simulink model "test_on_proxy"  (R2025b)
settings: Solver=FixedStepAuto  StartTime=0.0  StopTime=91  FixedStep=0.001  RelTol=1e-3
undefined symbols (not defined in the file): DiscIntNeverNeededParam, Ts, x0_eq
libraries: eeGeneralControl x1
(part 1 of 2)
settings Model: Creator=Juuzo  LastModifiedBy=Juuzo
settings SolverCC: AlgebraicLoopSolver=TrustRegion
settings SFSimCC: CustomCodeUndefinedFunction=UseInterfaceOnly
settings RTWCC: GPUComputeCapability=3.5

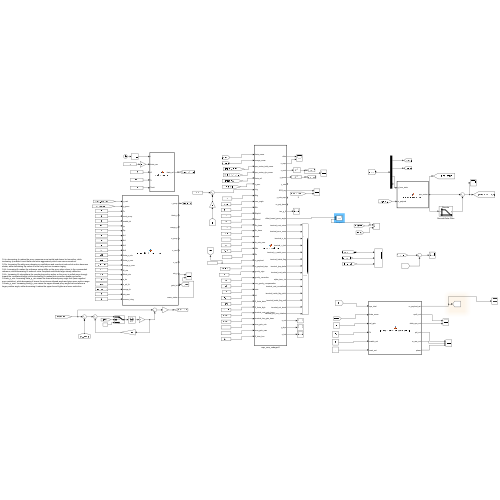
[thumbnail: Simulink's stored preview of the top-level diagram]
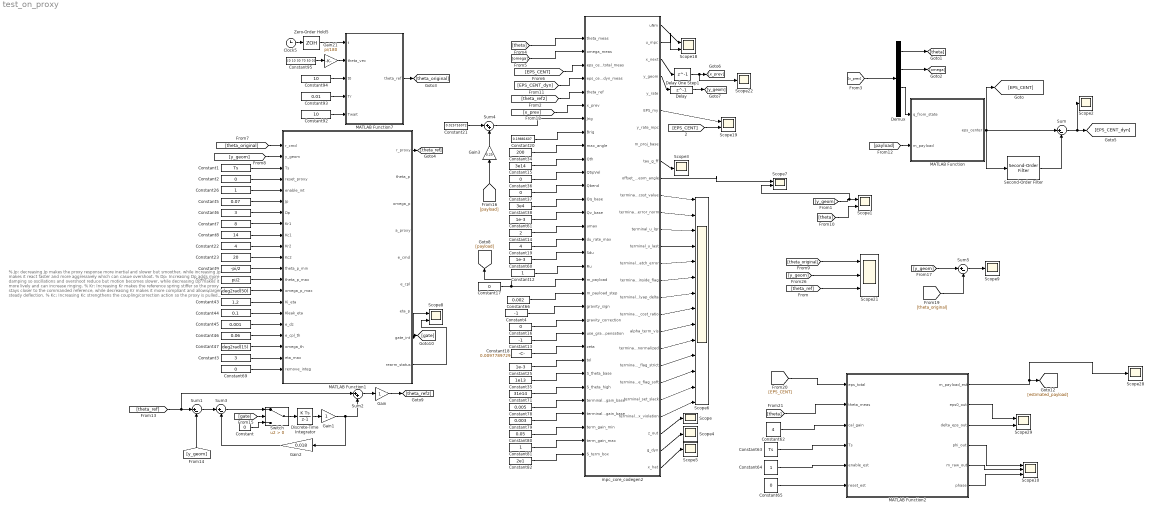
== system test_on_proxy ==
  note: % Jp: decreasing Jp makes the proxy response more inertial and slower but smoother, while increasing Jp makes it react faster and more aggressively which can casue overshoot.
      | % Dp: Increasing Dp adds more damping so oscillations and overshoot reduce but motion becomes slower, while decreasing Dp makes it more lively and can increase ringing.
      | % Kr: Increasing Kr makes the reference spring stiffer so the proxy stays closer to the commanded reference, while decreasing Kr makes it more compliant and allows larger steady deflection.
      | % Kc: Increasing Kc strengthens the coupling/correction action so the proxy is pulled more strongly toward the constrained target, while decreasing Kc makes that correction weaker and softer.
      | % theta_p_min: Increasing theta_p_min raises the lower allowed proxy angle limit (less negative / more restrictive), while decreasing it lowers the minimum allowed angle and gives more motion range.
      | % theta_p_max: Increasing theta_p_max raises the upper allowed proxy angle limit and allows a larger positive angle, while decreasing it makes the upper bound tighter and more restrictive.
  Clock5 : Clock
  Constant{,2,16..17,37,65,69} (7 alike) : Constant  Value=0
  Constant1 : Constant  Value=Ts
  Constant10 : Constant  Value=deg2rad(50)
  Constant11 : Constant  Value=pi/2
  Constant12 : Constant
  Constant13 : Constant  Value=-1
  Constant14 : Constant  Value=2
  Constant15 : Constant  Value=3e14  VectorParams1D=off
  Constant18 : Constant  Value=0.0097789729
  Constant19 : Constant  Value=4
  Constant20 : Constant  Value=0.19881607
  Constant21 : Constant  Value=0.025755072
  Constant22 : Constant  Value=4
  Constant23 : Constant  Value=20
  Constant25 : Constant  Value=1e-3
  Constant26 : Constant  VectorParams1D=off
  Constant3 : Constant  Value=3
  Constant34 : Constant  Value=200
  Constant35 : Constant  Value=1e13
  Constant36 : Constant  Value=0  VectorParams1D=off
  Constant38 : Constant  Value=3e4  VectorParams1D=off
  Constant4 : Constant  Value=-1
  Constant43 : Constant  Value=1.2
  Constant44 : Constant  Value=0.1
  Constant45 : Constant  Value=0.001
  Constant46 : Constant  Value=0.06
  Constant47 : Constant  Value=deg2rad(15)
  Constant5 : Constant  Value=0.07
  Constant6 : Constant  Value=3
  Constant60 : Constant  Value=1e-3
  Constant61 : Constant  Value=1e-3
  Constant62 : Constant  Value=4
  Constant63 : Constant  Value=Ts
  Constant64 : Constant
  Constant66 : Constant  Value=0.002
  Constant7 : Constant  Value=8
  Constant71 : Constant  Value=31e14
  Constant78 : Constant  Value=0.005
  Constant79 : Constant  Value=0.003
  Constant8 : Constant  Value=14
  Constant80 : Constant  Value=0.05
  Constant81 : Constant
  Constant82 : Constant  Value=2e1
  Constant9 : Constant  Value=-pi/2
  Constant92 : Constant  Value=10
  Constant93 : Constant  Value=0.01
  Constant94 : Constant  Value=10
  Constant95 : Constant  Value=[0 10 30 70 50 0]  VectorParams1D=off
  Delay : Delay  DelayLength=1
  Delay One Step1 : Delay  DelayLength=1  InitialCondition=[-0.4 0 0 0]  SampleTime=Ts
  Demux : Demux  Outputs=size(x0_eq,1)
  Discrete-Time Integrator : DiscreteIntegrator  SampleTime=-1  ICPrevOutput=DiscIntNeverNeededParam  ICPrevScaledInput=DiscIntNeverNeededParam
  Gain : Gain
  Gain1 : Gain
  Gain2 : Gain  Gain=0.018
  Gain21 : Gain  Gain=pi/180
  Gain3 : Gain  Gain=0.25
  MATLAB Function : MATLAB Function  TreatAsAtomicUnit=on
  MATLAB Function1 : MATLAB Function  TreatAsAtomicUnit=on
  MATLAB Function2 : MATLAB Function  TreatAsAtomicUnit=on  SystemSampleTime=0.001
  MATLAB Function7 : MATLAB Function  TreatAsAtomicUnit=on
  Scope{,2..5,9,22,28} (8 alike) : Scope
      Scope settings: ActiveDisplayYMinimum=0.03462626429758181  ActiveDisplayYMaximum=0.14630000608700439
      Scope2 settings: ActiveDisplayYMinimum=-2.6432719878301515E-6  ActiveDisplayYMaximum=1.0572577019271434E-6  DataLoggingVariableName=ScopeData2
      Scope22 settings: ActiveDisplayYMinimum=-0.0014754347139640661  ActiveDisplayYMaximum=0.0005793847718010294  DataLoggingVariableName=ScopeData7
      Scope28 settings: ActiveDisplayYMinimum=-0.00425  ActiveDisplayYMaximum=0.03825  DataLoggingVariableName=ScopeData15
      Scope3 settings: ActiveDisplayYMinimum=-1  ActiveDisplayYMaximum=1  DataLoggingVariableName=ScopeData5
      Scope4 settings: ActiveDisplayYMinimum=0.03462626429758181  ActiveDisplayYMaximum=0.14630000608700439  DataLoggingVariableName=ScopeData8
      Scope5 settings: ActiveDisplayYMinimum=0.03462626429758181  ActiveDisplayYMaximum=0.14630000608700439  DataLoggingVariableName=ScopeData9
      Scope9 settings: ActiveDisplayYMinimum=-0.00729154121661256  ActiveDisplayYMaximum=0.005693566274452444  DataLoggingVariableName=ScopeData13
  Scope{1,7..8,18..19,29} (6 alike) : Scope  NumInputPorts=2
      Scope1 settings: ActiveDisplayYMinimum=-1  ActiveDisplayYMaximum=1
      Scope18 settings: ActiveDisplayYMinimum=-2.5  ActiveDisplayYMaximum=2.5  DataLoggingVariableName=ScopeData3
      Scope19 settings: ActiveDisplayYMinimum=-4.4042134344337806E+284  ActiveDisplayYMaximum=1.9921108400400171E+284  DataLoggingVariableName=ScopeData4
      Scope29 settings: ActiveDisplayYMinimum=6.3875  ActiveDisplayYMaximum=6.5125  DataLoggingVariableName=ScopeData16
      Scope7 settings: ActiveDisplayYMinimum=-0.00025935118136851537  ActiveDisplayYMaximum=0.007136419000205705  DataLoggingVariableName=ScopeData11
      Scope8 settings: ActiveDisplayYMinimum=-0.12499999999999997  ActiveDisplayYMaximum=1.125  DataLoggingVariableName=ScopeData12
  Scope10 : Scope  NumInputPorts=3
      settings: ActiveDisplayYMinimum=-0.06335  ActiveDisplayYMaximum=0.08278  DataLoggingVariableName=ScopeData14
  Scope21 : Scope  NumInputPorts=3
      settings: ActiveDisplayYMinimum=-0.60273685089963092  ActiveDisplayYMaximum=1.4244490683177709  DataLoggingVariableName=ScopeData6
  Scope6 : Scope  NumInputPorts=14
      settings: ActiveDisplayYMinimum=-1  ActiveDisplayYMaximum=1  DataLoggingVariableName=ScopeData10
  Second-Order Filter : eeGeneralControl/Second-Order Filter  FilterType=Low-pass  fn=25  Zeta=0.707  Ts=-1  A0=0  Ph0=0  f0=0  b0=0
      settings: LibrarySourceBlock=ee_sl_lib/General Control/Second-Order Filter
  Sum{,1,3,5} (4 alike) : Sum  Inputs=|+-
  Sum2 : Sum  Inputs=|++
  Sum4 : Sum  Inputs=|++
  Switch : Switch  Criteria=u2 > Threshold  SaturateOnIntegerOverflow=off  InputSameDT=off
  Zero-Order Hold5 : ZeroOrderHold  SampleTime=Ts
  mpc_core_codegen2 : MATLAB Function  TreatAsAtomicUnit=on  SystemSampleTime=Ts
  wires:
  [x_prev] -> Demux/1
  Constant93/1 -> MATLAB Function7/4(Tr)
  Gain21/1 -> MATLAB Function7/2(theta_vec)
  Zero-Order Hold5/1 -> MATLAB Function7/1(t)
  Clock5/1 -> Zero-Order Hold5/1
  Constant94/1 -> MATLAB Function7/3(t0)
  Constant92/1 -> MATLAB Function7/5(Twait)
  [EPS_CENT] -> Scope19/2
  Constant95/1 -> Gain21/1
  [theta_original] -> MATLAB Function1/1(r_cmd)
  [y_geom] -> MATLAB Function1/2(y_geom)
  MATLAB Function7/1(theta_ref) -> [theta_original]
  MATLAB Function1/1(r_proxy) -> [theta_ref]
  Demux/3 -> MATLAB Function/1(q_from_state)
  Demux/1 -> [theta]
  Demux/2 -> [omega]
  MATLAB Function/1(eps_center) -> Second-Order Filter/1, Sum/1, [EPS_CENT]
  Delay/1 -> [y_geom]
  [theta_original] -> Scope21/1
  [theta_ref] -> Scope21/3
  Delay One Step1/1 -> Scope22/1, [x_prev]
  [y_geom] -> Scope21/2
  [y_geom] -> Scope7/2, Scope1/1
  [theta] -> Scope1/2
  [theta] -> mpc_core_codegen2/1(theta_meas)
  [omega] -> mpc_core_codegen2/2(omega_meas)
  [EPS_CENT] -> mpc_core_codegen2/3(eps_center_total_meas)
  Constant20/1 -> mpc_core_codegen2/8(Brig)
  [x_prev] -> mpc_core_codegen2/6(x_prev)
  [theta_ref2] -> mpc_core_codegen2/5(theta_ref)
  Second-Order Filter/1 -> Sum/2
  Sum/1 -> Scope2/1, [EPS_CENT_dyn]
  mpc_core_codegen2/1(uNm) -> Scope18/1
  mpc_core_codegen2/2(u_mpc) -> Scope18/2
  mpc_core_codegen2/3(x_next) -> Delay One Step1/1
  mpc_core_codegen2/4(y_geom) -> Delay/1
  [payload] -> MATLAB Function/2(m_payload)
  mpc_core_codegen2/6(EPS_my) -> Scope19/1
  mpc_core_codegen2/9(tau_g_ff) -> Scope3/1
  mpc_core_codegen2/25(z_out) -> Scope/1
  mpc_core_codegen2/26(g_dyn) -> Scope4/1
  mpc_core_codegen2/27(x_hat) -> Scope5/1
  mpc_core_codegen2/10(offset_based_geom_angle) -> Scope7/1
  mpc_core_codegen2/11(terminal_cost_value) -> Scope6/1
  mpc_core_codegen2/12(terminal_error_norm) -> Scope6/2
  mpc_core_codegen2/13(terminal_u_lqr) -> Scope6/3
  mpc_core_codegen2/14(terminal_u_last) -> Scope6/4
  mpc_core_codegen2/15(terminal_u_match_error) -> Scope6/5
  mpc_core_codegen2/16(terminal_inside_flag) -> Scope6/6
  mpc_core_codegen2/17(terminal_lyap_delta) -> Scope6/7
  mpc_core_codegen2/18(terminal_cost_ratio) -> Scope6/8
  mpc_core_codegen2/19(alpha_term_vis) -> Scope6/9
  mpc_core_codegen2/20(terminal_cost_normalized) -> Scope6/10
  mpc_core_codegen2/21(terminal_inside_flag_strict) -> Scope6/11
  mpc_core_codegen2/22(terminal_inside_flag_soft) -> Scope6/12
  mpc_core_codegen2/23(terminal_set_slack) -> Scope6/13
  mpc_core_codegen2/24(terminal_set_box_violation) -> Scope6/14
  [theta_ref] -> Sum2/1, Sum1/1
  [y_geom] -> Sum1/2
  Sum2/1 -> Gain/1
  Gain/1 -> [theta_ref2]
  [gate] -> Switch/2
  MATLAB Function1/8(gate_int) -> [gate], Scope8/1
  Constant/1 -> Switch/3
  Sum1/1 -> Sum3/1
  Sum3/1 -> Switch/1
  Switch/1 -> Discrete-Time Integrator/1
  Discrete-Time Integrator/1 -> Gain1/1
  Gain1/1 -> Sum2/2, Gain2/1
  Gain2/1 -> Sum3/2
  Constant21/1 -> Sum4/1
  [payload] -> Gain3/1
  Sum4/1 -> mpc_core_codegen2/7(Jrig)
  Gain3/1 -> Sum4/2
  MATLAB Function1/9(rearm_status) -> Scope8/2
  [y_geom] -> Sum5/1
  [theta_original] -> Sum5/2
  Sum5/1 -> Scope9/1
  [EPS_CENT_dyn] -> mpc_core_codegen2/4(eps_center_dyn_meas)
  Constant63/1 -> MATLAB Function2/4(Ts)
  MATLAB Function2/6(phase) -> Scope10/3
  [theta] -> MATLAB Function2/2(theta_meas)
  MATLAB Function2/4(phi_out) -> Scope10/1
  [EPS_CENT] -> MATLAB Function2/1(eps_total)
  Constant65/1 -> MATLAB Function2/6(reset_est)
  MATLAB Function2/5(m_raw_out) -> Scope10/2
  MATLAB Function2/3(delta_eps_out) -> Scope29/2
  MATLAB Function2/2(eps0_out) -> Scope29/1
  MATLAB Function2/1(m_payload_est) -> Scope28/1, [estimated_payload]
  Constant64/1 -> MATLAB Function2/5(enable_est)
  Constant62/1 -> MATLAB Function2/3(cal_gain)
  Constant12/1 -> mpc_core_codegen2/18(Ru)
  Constant36/1 -> mpc_core_codegen2/11(QtipVel)
  Constant13/1 -> mpc_core_codegen2/23(use_gravity_compensation)
  Constant71/1 -> mpc_core_codegen2/27(S_theta_high)
  Constant25/1 -> mpc_core_codegen2/25(tol)
  Constant79/1 -> mpc_core_codegen2/29(terminal_law_gain_base)
  Constant15/1 -> mpc_core_codegen2/10(Qth)
  Constant60/1 -> mpc_core_codegen2/17(Sdu)
  Constant66/1 -> mpc_core_codegen2/20(m_payload_step)
  Constant78/1 -> mpc_core_codegen2/28(terminal_cost_gain_base)
  Constant38/1 -> mpc_core_codegen2/13(Qq_base)
  Constant4/1 -> mpc_core_codegen2/21(gravity_sign)
  Constant16/1 -> mpc_core_codegen2/22(gravity_correction)
  Constant18/1 -> mpc_core_codegen2/24(zeta)
  Constant80/1 -> mpc_core_codegen2/30(term_gain_min)
  Constant35/1 -> mpc_core_codegen2/26(S_theta_base)
  Constant19/1 -> mpc_core_codegen2/16(du_rate_max)
  Constant14/1 -> mpc_core_codegen2/15(umax)
  Constant61/1 -> mpc_core_codegen2/14(Qv_base)
  Constant34/1 -> mpc_core_codegen2/9(max_angle)
  Constant37/1 -> mpc_core_codegen2/12(Qbend)
  Constant82/1 -> mpc_core_codegen2/32(S_term_box)
  Constant81/1 -> mpc_core_codegen2/31(term_gain_max)
  Constant17/1 -> mpc_core_codegen2/19(m_payload), [payload]
  Constant7/1 -> MATLAB Function1/8(Kr1)
  Constant46/1 -> MATLAB Function1/18(e_cpl_th)
  Constant8/1 -> MATLAB Function1/9(Kc1)
  Constant10/1 -> MATLAB Function1/14(omega_p_max)
  Constant9/1 -> MATLAB Function1/12(theta_p_min)
  Constant23/1 -> MATLAB Function1/11(Kc2)
  Constant11/1 -> MATLAB Function1/13(theta_p_max)
  Constant47/1 -> MATLAB Function1/19(omega_th)
  Constant26/1 -> MATLAB Function1/5(enable_int)
  Constant44/1 -> MATLAB Function1/16(Kleak_eta)
  Constant2/1 -> MATLAB Function1/4(reset_proxy)
  Constant22/1 -> MATLAB Function1/10(Kr2)
  Constant1/1 -> MATLAB Function1/3(Ts)
  Constant5/1 -> MATLAB Function1/6(Jp)
  Constant43/1 -> MATLAB Function1/15(Ki_eta)
  Constant3/1 -> MATLAB Function1/20(eta_max)
  Constant69/1 -> MATLAB Function1/21(remove_integ)
  Constant45/1 -> MATLAB Function1/17(e_dz)
  Constant6/1 -> MATLAB Function1/7(Dp)

== matlab function test_on_proxy/MATLAB Function1 ==
  data: r_cmd input; r_proxy output; y_geom input; Ts input; reset_proxy input; enable_int input; Jp input; Dp input; Kr1 input; Kc1 input; Kr2 input; Kc2 input; theta_p_min input; theta_p_max input; omega_p_max input; theta_p output; omega_p output; a_proxy output; e_cmd output; e_cpl output; Ki_eta input; Kleak_eta input; e_dz input; e_cpl_th input; omega_th input; eta_max input; eta_p output; gate_int output; remove_integ input; rearm_status output
function [r_proxy, theta_p, omega_p, a_proxy, e_cmd, e_cpl, eta_p, gate_int,rearm_status] = proxy_virtual_beam_int_strict( ...
    r_cmd, y_geom, Ts, reset_proxy, enable_int, ...
    Jp, Dp, Kr1, Kc1, Kr2, Kc2, ...
    theta_p_min, theta_p_max, omega_p_max, ...
    Ki_eta, Kleak_eta, e_dz, e_cpl_th, omega_th, eta_max,remove_integ) %#codegen

persistent thp wpp etap init_done
persistent int_armed
persistent r_cmd_prev
persistent soft_mode
persistent abs_e_prev err_dec_count
persistent e_bias_prev

if isempty(init_done)
    thp = 0.0;
    wpp = 0.0;
    etap = 0.0;
    int_armed = 1.0;
    r_cmd_prev = r_cmd;
    soft_mode = 0.0;
    abs_e_prev = 0.0;
    err_dec_count = 0.0;
    e_bias_prev = 0.0;
    init_done = true;
end

if reset_proxy ~= 0
    thp  = 0.0;
    wpp  = 0.0;
    etap = 0.0;
    int_armed = 1.0;
    r_cmd_prev = r_cmd;
    soft_mode = 0.0;
    abs_e_prev = 0.0;
    err_dec_count = 0.0;
    e_bias_prev = 0.0;
end

Ts_eff      = max(Ts, 1e-9);
Jp_eff      = max(Jp, 1e-9);
wmax        = max(omega_p_max, 1e-9);
eta_lim     = max(abs(eta_max), 1e-9);

e_dead      = max(abs(e_dz), 0.0);
e_act       = max(abs(e_cpl_th), e_dead + 1e-9);

% smarter / earlier rearm than previous 2.0*e_act
e_rearm     = 1.2 * e_act;

omega_lim   = max(abs(omega_th), 0.0);

% -------------------------------------------------------------------------
% command-change detection
% if original reference changes, leave soft mode immediately
% -------------------------------------------------------------------------
r_move_th = 0.1*pi/180.0;
r_changed = abs(r_cmd - r_cmd_prev) >= r_move_th;
r_is_static = ~r_changed;

if r_changed
    soft_mode = 0.0;
    int_armed = 1.0;
    err_dec_count = 0.0;
    e_bias_prev = 0.0;
end

% -------------------------------------------------------------------------
% current coupling error between proxy and real beam
% positive if proxy is ahead of the real beam
% -------------------------------------------------------------------------
e_cpl_k = thp - y_geom;

% -------------------------------------------------------------------------
% bias error for integral action
% -------------------------------------------------------------------------
e_bias = r_cmd - y_geom;
abs_e_bias = abs(e_bias);

% -------------------------------------------------------------------------
% release detection while in soft mode
% if error is decreasing for several samples, assume beam was released
% and return to normal stiffness so it comes back faster
% -------------------------------------------------------------------------
N_dec_required = 10.0;
e_dec_tol = 0.02*pi/180.0;

if soft_mode ~= 0.0
    if abs_e_bias < (abs_e_prev - e_dec_tol)
        err_dec_count = err_dec_count + 1.0;
    else
        err_dec_count = 0.0;
    end

    if err_dec_count >= N_dec_required
        soft_mode = 0.0;
        err_dec_count = 0.0;
    end
else
    err_dec_count = 0.0;
end

abs_e_prev = abs_e_bias;

% -------------------------------------------------------------------------
% smarter integral arming logic
%
% old problem:
%   if error entered deadzone during overshoot, integral was disarmed
%   and stayed off until abs(error) reached a large rearm threshold.
%
% new idea:
%   disarm only if close to reference AND not moving away.
%   if error crossed sign or starts growing again, keep/rearm integral.
% -------------------------------------------------------------------------
e_dot_est = (e_bias - e_bias_prev) / Ts_eff;

% true if error magnitude is increasing
moving_away = (e_bias * e_dot_est) > 0.0;

% true if beam crossed the reference
sign_crossed = (e_bias * e_bias_prev) < 0.0;

if abs_e_bias <= e_dead
    if moving_away || sign_crossed
        int_armed = 1.0;
    else
        int_armed = 0.0;
    end
elseif abs_e_bias >= e_act
    int_armed = 1.0;
end
rearm_status = int_armed;
% -------------------------------------------------------------------------
% final strict integral gate
% allow integral action up to e_rearm for overshoot recovery
% -------------------------------------------------------------------------
if (enable_int ~= 0) && ...
   (int_armed ~= 0) && ...
   (abs_e_bias > e_dead) && ...
   (abs_e_bias <= e_rearm) && ...
   (abs(wpp) <= omega_lim)
    gate = 1.0;
else
    gate = 0.0;
end

% -------------------------------------------------------------------------
% latch soft/compliant mode
%
% enter soft mode only when:
%   1) command is constant
%   2) beam is fully close to reference, inside deadband
%   3) proxy is moving slowly
%   4) integral gate is already off
%
% once soft_mode = 1, keep it no matter gate changes,
% until r_cmd changes or release detection switches it back.
% -------------------------------------------------------------------------
near_dead  = abs_e_bias <= e_dead;
proxy_slow = abs(wpp) <= omega_lim;

if (soft_mode == 0.0) && r_is_static && near_dead && proxy_slow && (gate == 0.0)
    soft_mode = 1.0;
end

if soft_mode ~= 0.0
    Kr_eff = Kr2;
    Kc_eff = Kc2;
else
    Kr_eff = Kr1;
    Kc_eff = Kc1;
end

e_bias_dz = deadzone_scalar(e_bias, e_dead);

% -------------------------------------------------------------------------
% internal integral bias state
% if gate = 0, eta is frozen
% -------------------------------------------------------------------------
if gate ~= 0
    eta_dot = Ki_eta * e_bias_dz - Kleak_eta * etap;
else
    eta_dot = 0.0;
end

etap = etap + Ts_eff * eta_dot;
etap = clamp_scalar(etap, -eta_lim, eta_lim);

% -------------------------------------------------------------------------
% command-side spring error
% -------------------------------------------------------------------------
e_cmd_k = (r_cmd + remove_integ*etap) - thp;

% -------------------------------------------------------------------------
% proxy rigid-body dynamics
% -------------------------------------------------------------------------
w_dot = (-Dp*wpp + Kr_eff*e_cmd_k - Kc_eff*e_cpl_k) / Jp_eff;

wpp = wpp + Ts_eff * w_dot;
wpp = clamp_scalar(wpp, -wmax, wmax);

thp = thp + Ts_eff * wpp;
thp = clamp_scalar(thp, theta_p_min, theta_p_max);

if (thp <= theta_p_min) && (wpp < 0.0)
    wpp = 0.0;
elseif (thp >= theta_p_max) && (wpp > 0.0)
    wpp = 0.0;
end

% update memories
r_cmd_prev = r_cmd;
e_bias_prev = e_bias;

r_proxy  = thp;
theta_p  = thp;
omega_p  = wpp;
a_proxy  = w_dot;
e_cmd    = e_cmd_k;
e_cpl    = e_cpl_k;
eta_p    = etap;
gate_int = gate;

end

function y = clamp_scalar(x, xmin, xmax)
y = min(max(x, xmin), xmax);
end

function y = deadzone_scalar(x, dz)
if abs(x) <= dz
    y = 0.0;
elseif x > dz
    y = x - dz;
else
    y = x + dz;
end
end

== matlab function test_on_proxy/MATLAB Function ==
  data: q_from_state input; eps_center output; m_payload input
function eps_center = eps_from_state_block(q_from_state, m_payload)
%#codegen
% Standalone strain generator from modal state q1
%
% Input:
%   q_from_state : modal coordinate q1
%   m_payload    : payload mass at beam tip [kg]
%
% Output:
%   eps_center   : strain at sensor location
%
% Assumption:
%   payload rotational inertia J_tip = 0

persistent init_done last_m_payload k_strain

% --- required explicit initialization for MATLAB Function/codegen ---
if isempty(init_done)
    init_done = false;
    last_m_payload = 0.0;
    k_strain = 0.0;
end

need_rebuild = false;
if ~init_done
    need_rebuild = true;
elseif abs(last_m_payload - m_payload) > 1e-12
    need_rebuild = true;
end

if need_rebuild

    % ===== geometry & material =====
    L   = 0.5;
    b   = 0.02;
    h   = 0.002;
    E   = 70e9;
    rho = 2755;

    Acs  = b*h;
    Izz  = b*h^3/12;
    rhoA = rho*Acs;
    yb   = 0.5*h;

    % ===== payload =====
    M_tip = m_payload;
    J_tip = 0.0;

    % ===== spatial grid for normalization =====
    Ns = 100;
    s  = linspace(0, L, Ns).';

    w_trap = zeros(Ns,1);
    for i = 2:Ns
        hseg = s(i) - s(i-1);
        w_trap(i-1) = w_trap(i-1) + 0.5*hseg;
        w_trap(i)   = w_trap(i)   + 0.5*hseg;
    end

    % ===== first payload-aware root lambda = betaL =====
    betaL = compute_first_payload_root(rhoA, L, M_tip, J_tip);

    % ===== payload-aware shape =====
    phi_raw_tip = payload_shape_local(betaL, L, L, rhoA, M_tip);
    sc = 1 / max(abs(phi_raw_tip), 1e-12);

    phi_raw  = payload_shape_local(betaL, L, s, rhoA, M_tip) * sc;
    dphi_raw = payload_shape_d_local(betaL, L, s, rhoA, M_tip) * sc;

    % ===== payload-aware modal mass normalization =====
    mi = dot(w_trap, rhoA * (phi_raw.^2)) ...
       + M_tip * (phi_raw(end)^2) ...
       + J_tip * (dphi_raw(end)^2);

    cn = 1 / sqrt(max(mi, 1e-12));

    % ===== strain coefficient at sensor =====
    sensor_s = 0.05;

    phi_dd_i = payload_shape_dd_local(betaL, L, sensor_s, rhoA, M_tip);
    phi_dd_i = phi_dd_i * sc;

    psi_dd_i = cn * phi_dd_i;

    % epsilon = yb * psi_dd * q
    k_strain = yb * psi_dd_i;

    last_m_payload = m_payload;
    init_done = true;
end

eps_center = k_strain * q_from_state;

end

% ============================================================
% Helpers
% ============================================================

function betaL = compute_first_payload_root(rhoA, L, M_tip, J_tip)
% Finds first positive root of the payload-aware frequency equation
% in dimensionless variable lambda = beta * L

x_prev = 0.20;
f_prev = freq_eq_payload_lambda_local(x_prev, rhoA, L, M_tip, J_tip);

step = 0.02;
betaL = 1.875104068711961; % safe fallback

x = x_prev + step;
while x <= 10.0
    f_now = freq_eq_payload_lambda_local(x, rhoA, L, M_tip, J_tip);

    if isfinite(f_prev) && isfinite(f_now)
        if (f_prev * f_now) < 0
            betaL = bisect_payload_root_local(x_prev, x, rhoA, L, M_tip, J_tip);
            return;
        end
    end

    x_prev = x;
    f_prev = f_now;
    x = x + step;
end
end

function root = bisect_payload_root_local(a, b, rhoA, L, M_tip, J_tip)
fa = freq_eq_payload_lambda_local(a, rhoA, L, M_tip, J_tip);
fb = freq_eq_payload_lambda_local(b, rhoA, L, M_tip, J_tip);

if abs(fa) < 1e-12
    root = a;
    return;
end
if abs(fb) < 1e-12
    root = b;
    return;
end

for it = 1:80
    c = 0.5 * (a + b);
    fc = freq_eq_payload_lambda_local(c, rhoA, L, M_tip, J_tip);

    if abs(fc) < 1e-12 || abs(b - a) < 1e-10
        root = c;
        return;
    end

    if (fa * fc) < 0
        b = c;
        fb = fc;
    else
        a = c;
        fa = fc;
    end
end

root = 0.5 * (a + b);
end

function val = freq_eq_payload_lambda_local(lam, rhoA, L, M_tip, J_tip)
% Payload-aware frequency equation in dimensionless form:
%
% 1 + cos(lam)cosh(lam)
% - mu*lam*(sin(lam)cosh(lam) - cos(lam)sinh(lam))
% - nu*lam^3*(sin(lam)cosh(lam) + cos(lam)sinh(lam))
% + mu*nu*lam^4*(1 - cos(lam)cosh(lam)) = 0

mu = 0.0;
den_m = rhoA * L;
if den_m > 1e-18
    mu = M_tip / den_m;
end

nu = 0.0;
den_j = rhoA * L^3;
if den_j > 1e-18
    nu = J_tip / den_j;
end

c  = cos(lam);
s  = sin(lam);
ch = cosh(lam);
sh = sinh(lam);

val = (1 + c*ch) ...
    - mu * lam   * (s*ch - c*sh) ...
    - nu * lam^3 * (s*ch + c*sh) ...
    + mu * nu * lam^4 * (1 - c*ch);
end

function alpha = payload_alpha_local(betaL, rhoA, L, M_tip)
a = 0.0;
den = rhoA * L;
if den > 1e-18
    a = M_tip / den;
end

num  = sinh(betaL) - sin(betaL) + a*betaL*(cosh(betaL) - cos(betaL));
dena = cos(betaL) + cosh(betaL) + a*betaL*(sinh(betaL) - sin(betaL));

if abs(dena) < 1e-12
    if dena >= 0
        dena = 1e-12;
    else
        dena = -1e-12;
    end
end

alpha = num / dena;
end

function phi = payload_shape_local(betaL, L, s, rhoA, M_tip)
bs  = (betaL / L) .* s;
alp = payload_alpha_local(betaL, rhoA, L, M_tip);
phi = cosh(bs) - cos(bs) + alp * (sin(bs) - sinh(bs));
end

function dphi = payload_shape_d_local(betaL, L, s, rhoA, M_tip)
bs  = (betaL / L) .* s;
alp = payload_alpha_local(betaL, rhoA, L, M_tip);
dphi = (betaL / L) * (sinh(bs) + sin(bs) + alp * (cos(bs) - cosh(bs)));
end

function d2phi = payload_shape_dd_local(betaL, L, s, rhoA, M_tip)
bs  = (betaL / L) .* s;
alp = payload_alpha_local(betaL, rhoA, L, M_tip);
d2phi = (betaL / L)^2 * (cosh(bs) + cos(bs) - alp * (sin(bs) + sinh(bs)));
end

== matlab function test_on_proxy/MATLAB Function2 ==
  settings: updateMethod=DISCRETE
  data: eps_total input; theta_meas input; cal_gain input; m_payload_est output; eps0_out output; delta_eps_out output; phi_out output; m_raw_out output; phase output; Ts input; enable_est input; reset_est input
function [m_payload_est, eps0_out, delta_eps_out, phi_out, m_raw_out, phase] = ...
    payload_estimator_static_debug(eps_total, theta_meas,cal_gain, Ts, enable_est, reset_est) %#codegen

m_payload_est = 0.0;
eps0_out = 0.0;
delta_eps_out = 0.0;
phi_out = 0.0;
m_raw_out = 0.0;
phase = 0.0;

% Beam parameters
L = 0.5;
b = 0.02;
h = 0.002;
E = 70e9;
Izz = b*h^3/12.0;
EI = E*Izz;
yb = 0.5*h;
sensor_s = 0.05;
g = 9.81;

% Timing
baseline_ignore_time = 5.0;
baseline_end_time = 10.0;
payload_start_time = 10.1;

% Tuning
alpha_eps = 0.005;       % faster average
payload_quant = 0.001;
m_max = 1.0;

% Calibration gain
% cal_gain = 2.3;

persistent sample_count eps_avg eps0_sum eps0_count eps0_hold

if isempty(sample_count)
    sample_count = 0.0;
    eps_avg = 0.0;
    eps0_sum = 0.0;
    eps0_count = 0.0;
    eps0_hold = 0.0;
end

if reset_est ~= 0
    sample_count = 0.0;
    eps_avg = 0.0;
    eps0_sum = 0.0;
    eps0_count = 0.0;
    eps0_hold = 0.0;
end

if enable_est == 0
    return;
end

Ts_eff = max(Ts, 1e-9);
sample_count = sample_count + 1.0;
t_now = sample_count * Ts_eff;

% Average total strain
eps_avg = (1.0 - alpha_eps)*eps_avg + alpha_eps*eps_total;

if t_now < baseline_ignore_time
    phase = 0.5;
    eps0_out = eps0_hold;
    return;
end

% Learn zero-payload baseline
if t_now <= baseline_end_time
    eps0_sum = eps0_sum + eps_avg;
    eps0_count = eps0_count + 1.0;
    eps0_hold = eps0_sum / max(eps0_count, 1.0);

    phase = 1.0;
    eps0_out = eps0_hold;
    return;
end

eps0_out = eps0_hold;

if t_now < payload_start_time
    phase = 2.0;
    delta_eps_out = eps_avg - eps0_hold;
    return;
end

% Direct static payload estimate
delta_eps = eps_avg - eps0_hold;
phi = (yb * g * (L - sensor_s) / EI) * cos(theta_meas);

delta_eps_out = delta_eps;
phi_out = phi;

if abs(phi) < 1e-12
    m_raw = 0.0;
else
    m_raw = cal_gain * abs(delta_eps) / abs(phi);
end

if m_raw > m_max
    m_raw = m_max;
end

m_payload_est = payload_quant * round(m_raw / payload_quant);
m_raw_out = m_raw;
phase = 4.0;

end
